simulink model "FHSSwithGFSK"  (R2026a)
settings: Solver=FixedStepDiscrete  StopTime=0.5  FixedStep=5e-6
model workspace (MAT data in the model file):
  INC_IF = 134217728
  KFM = 5368709.12
  g = [8.76923448324e-10 9.75407126666e-10 1.08456496117e-09 1.20550944904e-09 1.33946408029e-09 1.48777387652e-09 1.65191687444e-09 1.83351663353e-09 2.03435585287e-09 2.25639118884e-09 2.50176937245e-09 2.77284473231e-09 ... (600 elements, 1x600)]
  sosB = [6.45184912909e-06  1.29036982582e-05  6.45184912909e-06  1  -1.9256177521  0.96299405095; 1  0  -1  1  -1.93528815535  0.979808675865; 1  -2  1  1  -1.95089313273  0.982852038739]
  sosL = [1.93545410516e-06  1.93545410516e-06  0  1  -0.975177876181  0; 1  2  1  1  -1.97455796353  0.975181747089]
libraries: commrandsrc3 x2, dspsigops x2, commchan3 x1, commsink2 x1, simulink x1
settings Model: Creator=MADHAV  LastModifiedBy=MADHAV

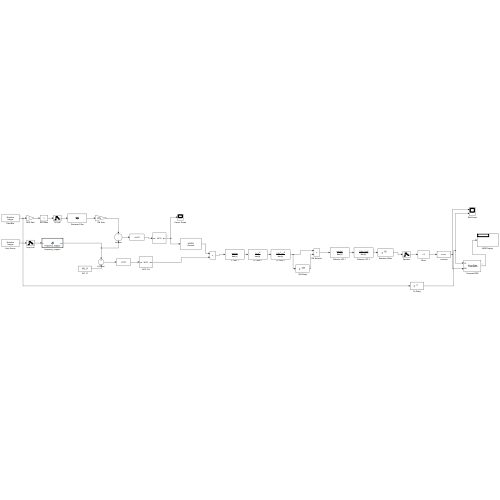
[thumbnail: Simulink's stored preview of the top-level diagram]
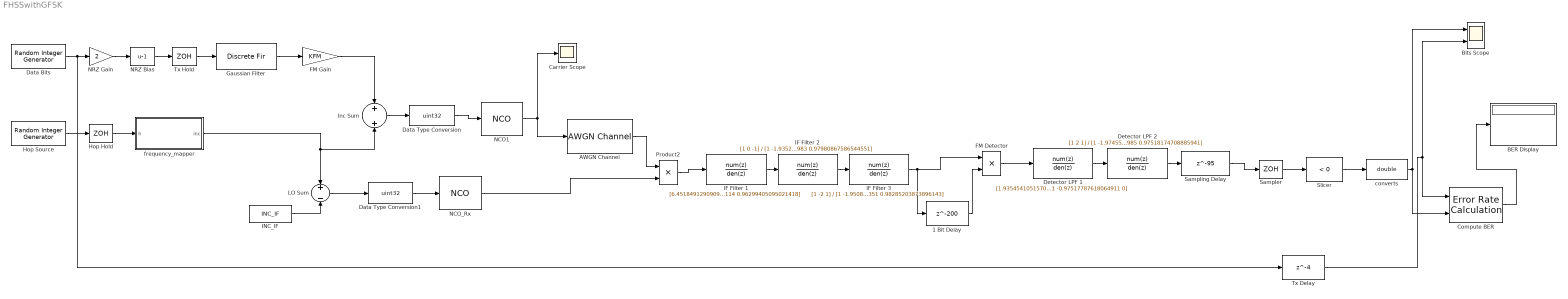
== system FHSSwithGFSK ==
  " converts" : DataTypeConversion  OutDataTypeStr=double  SaturateOnIntegerOverflow=off  RndMeth=Floor
  1 Bit Delay : Delay  DelayLength=200
  AWGN Channel : commchan3/AWGN Channel  LegacyMode=off  NoiseMethod="Signal to noise ratio  (SNR)"  noiseMode="Signal to noise ratio  (Eb/No)"  EbNo=10  EsNo=10  SNR=-10  BitsPerSymbol=1  SignalPower=1  SpecifySymbolPeriod=off  SamplesPerSymbol=200  SymbolPeriod=1  VarianceSource=Parameter  Variance=1  RandomStream=mt19937ar with seed  Seed=67  SimulateUsing=Interpreted execution
  BER Display : Display
  Bits Scope : Scope  NumInputPorts=2
      settings: ActiveDisplayYMinimum=0.33940201723534036  ActiveDisplayYMaximum=0.85440048376501454  DataLoggingVariableName=ScopeData3
  Carrier Scope : Scope
  Compute BER : commsink2/Error Rate Calculation  N=0  st_delay=20  cp_mode=Entire frame  subframe=[]  PMode=Port  WsName=ErrorVec  RsMode2=off  stop=off  numErr=100  maxBits=1e6
  Data Bits : commrandsrc3/Random Integer Generator  SetSize=2  SeedSource=Parameter  Seed=12345  SampleTime=1e-3  SamplesPerFrame=1  OutputDataType=double  SimulateUsing=Interpreted execution
  Data Type Conversion : DataTypeConversion  OutDataTypeStr=uint32  RndMeth=Nearest  SaturateOnIntegerOverflow=off
  Data Type Conversion1 : DataTypeConversion  OutDataTypeStr=uint32  RndMeth=Nearest  SaturateOnIntegerOverflow=off
  Detector LPF 1 : DiscreteFilter  Numerator=[1.9354541051570503e-06 1.9354541051570503e-06 0]  Denominator=[1 -0.97517787618064911 0]
  Detector LPF 2 : DiscreteFilter  Numerator=[1 2 1]  Denominator=[1 -1.9745579635256985 0.97518174708885941]
  FM Detector : Product
  FM Gain : Gain  Gain=KFM
  Gaussian Filter : DiscreteFir  Coefficients=g
  Hop Hold : ZeroOrderHold  SampleTime=5e-6
  Hop Source : commrandsrc3/Random Integer Generator  SetSize=37  SeedSource=Parameter  Seed=777  SampleTime=8e-3  SamplesPerFrame=1  OutputDataType=double  SimulateUsing=Interpreted execution
  IF Filter 1 : DiscreteFilter  Numerator=[6.4518491290909726e-06 1.2903698258181945e-05 6.4518491290909726e-06]  Denominator=[1 -1.9256177521002114 0.96299405095021418]
  IF Filter 2 : DiscreteFilter  Numerator=[1 0 -1]  Denominator=[1 -1.9352881553469983 0.97980867586544551]
  IF Filter 3 : DiscreteFilter  Numerator=[1 -2 1]  Denominator=[1 -1.9508931327307351 0.98285203873896143]
  INC_IF : Constant  Value=INC_IF
  Inc Sum : Sum
  LO Sum : Sum  Inputs=+-
  NCO1 : dspsigops/NCO  AccIncSrc=Input port  AccInc=100  PhaseOffsetSrc=Specify via dialog  PhaseOffset=0  AccumWL=32  HasDither=off  DitherWL=4  PNgeneratorLength=19  HasPhaseQuantizer=on  TableDepth=16  HasOutputPhaseError=off  Formula=Sine  DataType=double  OutputWL=16  OutputFL=14  CompMethod=Table lookup (no interpolation)  SampleTime=5e-6  SamplesPerFrame=1  OutputFrames=off
  NCO_Rx : dspsigops/NCO  AccIncSrc=Input port  AccInc=100  PhaseOffsetSrc=Specify via dialog  PhaseOffset=0  AccumWL=32  HasDither=off  DitherWL=4  PNgeneratorLength=19  HasPhaseQuantizer=on  TableDepth=16  HasOutputPhaseError=off  Formula=Sine  DataType=double  OutputWL=16  OutputFL=14  CompMethod=Table lookup (no interpolation)  SampleTime=5e-6  SamplesPerFrame=1  OutputFrames=off
  NRZ Bias : Bias  Bias=-1  SaturateOnIntegerOverflow=off
  NRZ Gain : Gain  Gain=2
  Product2 : Product
  Sampler : ZeroOrderHold  SampleTime=1e-3
  Sampling Delay : Delay  DelayLength=95
  Slicer : simulink/Logic and Bit Operations/Compare To Zero  relop=<  OutDataTypeStr=boolean
  Tx Delay : Delay  DelayLength=4
  Tx Hold : ZeroOrderHold  SampleTime=5e-6
  frequency_mapper : MATLAB Function  TreatAsAtomicUnit=on
  wires:
  IF Filter 1/1 -> IF Filter 2/1
  IF Filter 2/1 -> IF Filter 3/1
  Detector LPF 1/1 -> Detector LPF 2/1
  Data Bits/1 -> NRZ Gain/1, Tx Delay/1
  NRZ Gain/1 -> NRZ Bias/1
  NRZ Bias/1 -> Tx Hold/1
  Tx Hold/1 -> Gaussian Filter/1
  Gaussian Filter/1 -> FM Gain/1
  FM Gain/1 -> Inc Sum/1
  Hop Source/1 -> Hop Hold/1
  Hop Hold/1 -> frequency_mapper/1(h)
  frequency_mapper/1(inc) -> Inc Sum/2, LO Sum/1
  Inc Sum/1 -> Data Type Conversion/1
  Data Type Conversion/1 -> NCO1/1
  NCO1/1 -> AWGN Channel/1, Carrier Scope/1
  INC_IF/1 -> LO Sum/2
  LO Sum/1 -> Data Type Conversion1/1
  Data Type Conversion1/1 -> NCO_Rx/1
  AWGN Channel/1 -> Product2/1
  NCO_Rx/1 -> Product2/2
  Product2/1 -> IF Filter 1/1
  IF Filter 3/1 -> FM Detector/1, 1 Bit Delay/1
  1 Bit Delay/1 -> FM Detector/2
  FM Detector/1 -> Detector LPF 1/1
  Detector LPF 2/1 -> Sampling Delay/1
  Sampling Delay/1 -> Sampler/1
  Sampler/1 -> Slicer/1
  Slicer/1 -> " converts"/1
  Tx Delay/1 -> Bits Scope/2, Compute BER/1
  " converts"/1 -> Bits Scope/1, Compute BER/2
  Compute BER/1 -> BER Display/1

== matlab function FHSSwithGFSK/frequency_mapper ==
  data: h input; inc output
function inc = frequency_mapper(h) %#codegen
% hop index h = 0..36  ->  NCO phase increment (32-bit accumulator, Fs = 200 kHz)
% channels are 2 kHz apart starting at 10 kHz (time-scaled BLE: 1 MHz -> 1 kHz).  NOT rounded: the data is added before conversion.
f = 10e3 + 2e3*h;
inc = f*2^32/200000;
